simulink model "Clutch_Judder"  (R2024b)
settings: Solver=VariableStepAuto  StartTime=0.0  StopTime=10  RelTol=1e-3
values from neighbouring files (symbols this model uses):
  dt = 7.5    [Clutch_Judder_Para.m]
  dt1 = 1    [Clutch_Judder_Para.m]
  Iclutch = 5    [Clutch_Judder_Para.m]
  Ir = mv * r^2 / iA^2    (= 20)    [Clutch_Judder_Para.m]
  Kt = 1000    [Clutch_Judder_Para.m]
  Tclutch = 10    [Clutch_Judder_Para.m]
settings Model: Creator=dinul  LastModifiedBy=Dinulkar
settings RTWCC: GPUComputeCapability=3.5

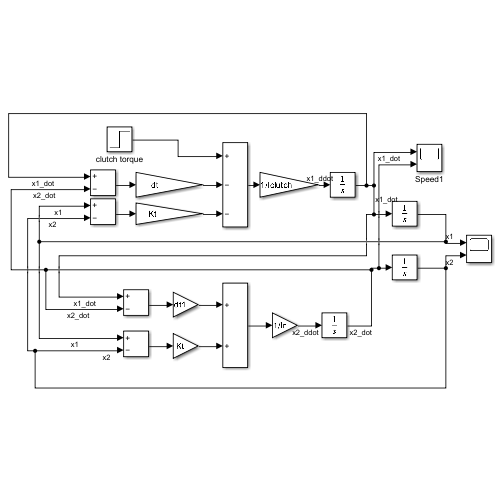
[thumbnail: Simulink's stored preview of the top-level diagram]
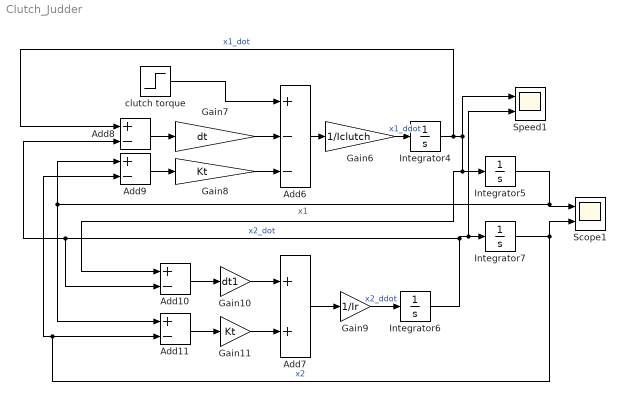
== system Clutch_Judder ==
  Add{8..11} (4 alike) : Sum  Inputs=+-
  Add6 : Sum  Inputs=+--
  Add7 : Sum
  Gain10 : Gain  Gain=dt1
  Gain11 : Gain  Gain=Kt
  Gain6 : Gain  Gain=1/Iclutch
  Gain7 : Gain  Gain=dt
  Gain8 : Gain  Gain=Kt
  Gain9 : Gain  Gain=1/Ir
  Integrator{4..7} (4 alike) : Integrator
  Scope1 : Scope  NumInputPorts=2
  Speed1 : Scope  NumInputPorts=2
  clutch torque : Step  After=Tclutch  SampleTime=0
  wires:
  clutch torque/1 -> Add6/1
  Gain7/1 -> Add6/2
  Add6/1 -> Gain6/1
  Gain6/1 -> Integrator4/1  "x1_ddot"
  Integrator7/1 -> Scope1/2, Add9/2, Add11/2  "x2"
  Integrator5/1 -> Add9/1, Add11/1, Scope1/1  "x1"
  Add10/1 -> Gain10/1
  Add11/1 -> Gain11/1
  Gain10/1 -> Add7/1
  Gain11/1 -> Add7/2
  Add7/1 -> Gain9/1
  Gain9/1 -> Integrator6/1  "x2_ddot"
  Integrator6/1 -> Integrator7/1, Speed1/2, Add10/2, Add8/2  "x2_dot"
  Add9/1 -> Gain8/1
  Add8/1 -> Gain7/1
  Gain8/1 -> Add6/3
  Integrator4/1 -> Add8/1, Speed1/1, Integrator5/1, Add10/1  "x1_dot"
